simulink model "w6_stage4_4_thermal_current"  (R2026a)
settings: Solver=ode45  StopTime=600  MaxStep=0.1  RelTol=1e-10  AbsTol=1e-12
settings Model: Creator=cogml  LastModifiedBy=cogml

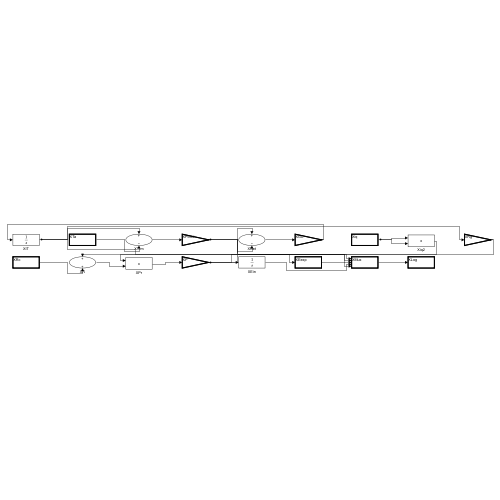
[thumbnail: Simulink's stored preview of the top-level diagram]
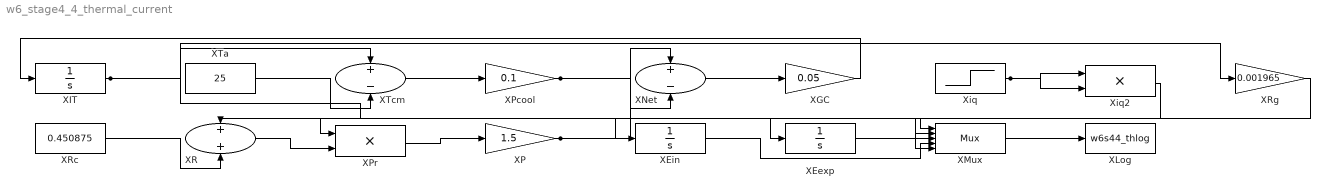
== system w6_stage4_4_thermal_current ==
  XEexp : Integrator
  XEin : Integrator
  XGC : Gain  Gain=0.05
  XIT : Integrator  InitialCondition=25
  XLog : ToWorkspace  VariableName=w6s44_thlog  SaveFormat=Timeseries  SampleTime=0.1
  XMux : Mux  Inputs=5
  XNet : Sum  Inputs=+-
  XP : Gain  Gain=1.5
  XPcool : Gain  Gain=0.1
  XPr : Product
  XR : Sum
  XRc : Constant  Value=0.450875
  XRg : Gain  Gain=0.001965
  XTa : Constant  Value=25
  XTcm : Sum  Inputs=+-
  Xiq : Step  Time=300  InitialValue=2  FinalValue=0  SampleTime=0
  Xiq2 : Product
  wires:
  XIT/1 -> XTcm/1, XRg/1, XMux/1
  XTa/1 -> XTcm/2
  XTcm/1 -> XPcool/1
  XNet/1 -> XGC/1
  XGC/1 -> XIT/1
  XPcool/1 -> XNet/2, XEexp/1, XMux/3
  Xiq/1 -> Xiq2/1, Xiq2/2
  XRg/1 -> XR/1
  XRc/1 -> XR/2
  Xiq2/1 -> XPr/1
  XR/1 -> XPr/2
  XPr/1 -> XP/1
  XP/1 -> XNet/1, XEin/1, XMux/2
  XEin/1 -> XMux/4
  XEexp/1 -> XMux/5
  XMux/1 -> XLog/1
